simulink model "KINvasion"  (Simulink 7.5)
settings: Solver=ode4  SolverMode=SingleTasking  StartTime=0.0  StopTime=inf  FixedStep=0.0005  RelTol=1e-3
model workspace (MAT data in the model file):
  col_x = 1
  col_y = 2
  EnemyNumber = 1
  DifficultyNumber = 2
  BaseRegen = 1
  WindowMinX = 2
  WindowMaxX = 3
  WindowMinY = 4
  WindowMaxY = 5
  ForceSize = 6
  FireTorque = 7
  MoneyPerShip = 9
  StartingMoney = 10
  StompForce = 8
  BombSize = 11
  MoneyDrops = 4
  BossNumber = 3
  DemoMode : num (value not decoded)
StartFcn:
  |  warndlg('Dexterit-E models cannot run under simulation. Please compile your model and run it from within Dexterit-E.');set_param(gcs,'SimulationCommand','stop')
undefined symbols (not defined in the file or in its folder): Process_Video_CMD, Video
libraries: xpclib x5, General x3, KINARM_general x1, KINARM_EP_loads x1
(part 1 of 3)
CloseFcn:
  | rtwprivate ssgencode ModelCloseRequest b2lab2d
settings Model: Creator=Chris Grebeldinger  LastModifiedBy=BrainAdjust  ModifiedComment=chris -- Wed Feb 16 09:18:30 2005 -- Version 1.1384  ModifiedHistory=Feb 16/05 - Add error repeat, add offset ramp  ExtModeArmWhenConnect=off  ExtModeLogAll=off  BufferReuse=off
settings SolverCC: AutoInsertRateTranBlk=on
settings DataIOCC: LimitDataPoints=off  SaveOutput=off  SaveTime=off  SignalLoggingName=sigsOut
settings OptimizationCC: BlockReduction=off  BooleanDataType=off  OptimizeBlockIOStorage=off  BufferReuse=off  EnforceIntegerDowncast=off  ExpressionFolding=off  FoldNonRolledExpr=off  LocalBlockOutputs=off  InitFltsAndDblsToZero=on
settings DebuggingCC: SaveWithParameterizedLinksMsg=none  SignalResolutionControl=TryResolveAllWithWarning  SolverPrmCheckMsg=none  MultiTaskDSMMsg=warning  MultiTaskCondExecSysMsg=none  StrictBusMsg=Warning
settings HardwareCC: ProdIntDivRoundTo=Zero  ProdEndianess=LittleEndian  ProdHWDeviceType=Generic->32-bit x86 compatible  TargetHWDeviceType=32-bit Generic
settings RTWCC: SystemTargetFile=xpctarget.tlc  TemplateMakefile=xpc_default_tmf  Description=xPC Target  ProcessScript=xpctarget_make_rtw_hook  IncludeERTFirstTime=on  RTWCompilerOptimization=On
settings CodeAppCC: MaxIdLength=63
settings xpcTargetCC: TargetFcnLib=ansi_tfl_tmw.mat  TargetFunctionLibrary=ANSI_C  ERTCodeCoverageTool=None  ParMdlRefBuildCompliant=off  PortableWordSizes=off  xPCisDownloadable=off  xPCLoadParamSetFile=off

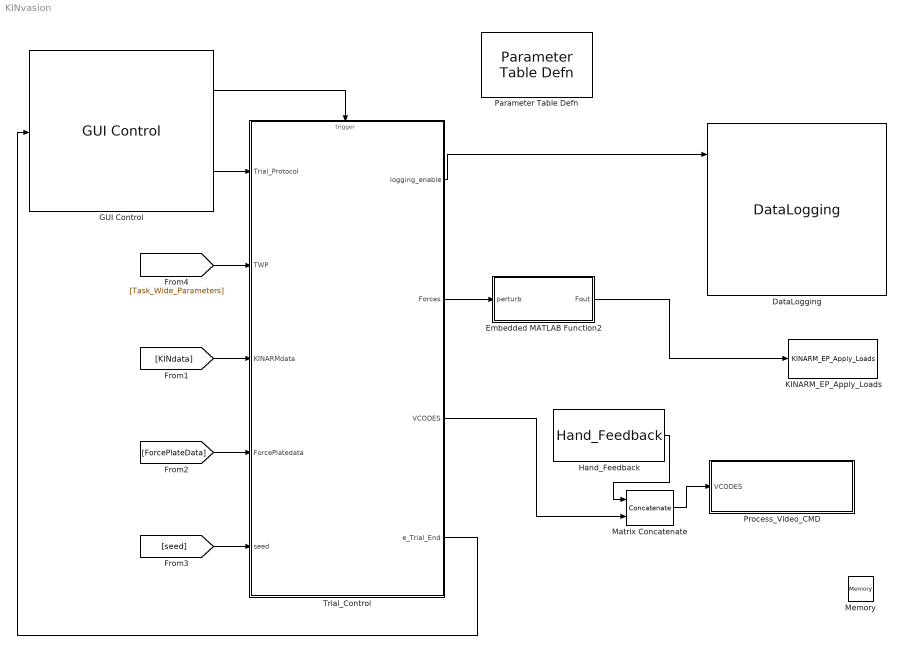
== system KINvasion ==
  DataLogging : General/DataLogging  SystemSampleTime=-1  log_event_codes=on  log_analog_inputs=on
      link override Poll KINARM/EPTorqueCMD: GotoTag=KINARMEPTorqueCMD
      link override Poll KINARM/TorqueCMD: GotoTag=KINARMTorqueCMD
  Embedded MATLAB Function2 : Stateflow chart  TreatAsAtomicUnit=on
  GUI Control : General/GUI Control  SystemSampleTime=-1  target_type_str=Circle  Target_Type=1  XYcols=[1 2]  Vcols=3  Lcols=4  indices_padding=[0 0 0 0;0 0 0 0]  task_version=1.0  show_repeat_trial_flag=off
  Hand_Feedback : KINARM_general/Hand_Feedback  SystemSampleTime=-1  feedback_cntl_src=none
  KINARM_EP_Apply_Loads : KINARM_EP_loads/KINARM_EP_Apply_Loads  SystemSampleTime=-1  up_duration=1500  down_duration=1500  max_force=30
  Matrix Concatenate : Concatenate  Mode=Multidimensional array
  Memory : Memory
  Parameter Table Defn : General/Parameter Table Defn  SystemSampleTime=-1  ShowInLibBrowser=0
  Process_Video_CMD : Subsystem  AncestorBlock=Video/Process_Video_CMD  LoadFcn=set_param(gcs, 'MaxIdLength', 63);  mask(Process_Video_CMD){}
      mask help:
      | <b>Do not rename this block, it must be called 'Process_Video_CMD'.</b>
      | <p>
      | This block takes a matrix of video commands (VCODES) as inputs (one VCODE per row) and processes them to display the appropriate video output.
      mask init:
      | block_path = gcb;  % store block path, as gcb may change with block operations
      | 
      | idxs = findstr(block_path, '/Process_Video_CMD');
      | [idxCount, n] = size(idxs);
      | [m, strlen] = size(block_path);
      | bColorSet = 0;
      | 
      | if idxCount == 0 || idxs(1) ~= strlen - 17
      |     fprintf('=========ERROR====================\n');
      |     fprintf('%s should be called Process_Video_CMD, attempting to rename.\n', block_path);
      |     try
      |         set_param(block_path, 'Name', 'Process_Video_CMD');
      |         block_path = gcb;  % store block path, as gcb may change with block operations
      |         fprintf('Rename successful\n');
      |     catch err
      |         fprintf('Rename failed. You may have 2 Process_Video_CMD blocks or another improperly named block.\n');
      |        	set_param(block_path, 'BackgroundColor', '[0.9, 0, 0]');
      |         bColorSet = 1;
      |     end
      |     fprintf('=============================\n');
      | end
      | 
      | 
      | % Handle background colours if link status changes.  If the link is resolved, 
      | % make the block back to the library colour.  If the link is not resolved, 
      | % change the colour to something other than the library block colour (but 
      | % only change it if it is the library colour, that way end-users can choose
      | % their own colour.
      | link_status = get_param(block_path, 'LinkStatus');
      | block_parent = get_param(block_path, 'Parent');
      | if bColorSet == 0 && (strcmp(link_status, 'resolved') || strcmp(block_parent, 'Video'))
      | 	set_param(block_path, 'BackgroundColor', '[0.85882, 0.69019, 0.3098]');
      | else
      |  	current_bgcolor = str2num( get_param(block_path, 'BackgroundColor') ) ;
      | 	%if the BackgroundColor is 'green', then after the str2num, current_bgcolor is empty
      | 	if ~isempty(current_bgcolor) 
      | 		if (round(current_bgcolor * 255) == [219 176 79])
      | 	 		set_param(block_path, 'BackgroundColor', 'green');
      | 		end
      | 	end
      | end
      mask Help:
      | Processes VCODES and sends a composite command over UDP to the GUI computer.
      | 
      | <H2>Library </H2>
      | Video
      | 
      | <H2>Description </H2>
      | <b>Do not rename this block, it must be called 'Process_Video_CMD'.</b>
      | <p>
      | The Process_Video_CMD block takes a matrix of video commands (VCODES) as inputs and processes them to display the appropriate video output.  The processed video command format is designed for use with GUI application.  There can be only one VCODE per row in the input.  To concatenate VCODEs properly prior to connecting a VCODE matrix to this block, the Matrix Concatenation block in the Simulink Math library should be used, with the concatenation method set to "Vertical".   For more information on the details of a VCODE, right click on the Show_Target block in the video library, click "Look Under Mask" and open the Embedded Matlab function.
      | <P>
      | The output command from this block is sent via UDP to an external computer for processing (note: this output is sent internally to the block - there is no output from the block that needs wiring to another block).
      | <P>
      | <B><I> There can be only one Process_Video_CMD block in a Task Program.</I></B>
      | 
      | <H2>Related Blocks </H2>
      | Show_Target<BR>
      | Show_Target_With_Label<BR>
      | Hand_Feedback<BR>
  Trial_Control : Stateflow chart  TreatAsAtomicUnit=on
  wires:
  GUI Control/2 -> Trial_Control/1(Trial_Protocol)
  GUI Control/1 -> Trial_Control/Trigger
  Trial_Control/1(logging_enable) -> DataLogging/1
  Trial_Control/4(e_Trial_End) -> GUI Control/1
  [Task_Wide_Parameters] -> Trial_Control/2(TWP)
  [KINdata] -> Trial_Control/3(KINARMdata)
  [seed] -> Trial_Control/5(seed)
  Trial_Control/3(VCODES) -> Matrix Concatenate/2
  Matrix Concatenate/1 -> Process_Video_CMD/1(VCODES)
  Hand_Feedback/1 -> Matrix Concatenate/1
  Embedded MATLAB Function2/1(Fout) -> KINARM_EP_Apply_Loads/1
  Trial_Control/2(Forces) -> Embedded MATLAB Function2/1(perturb)
  [ForcePlateData] -> Trial_Control/4(ForcePlatedata)

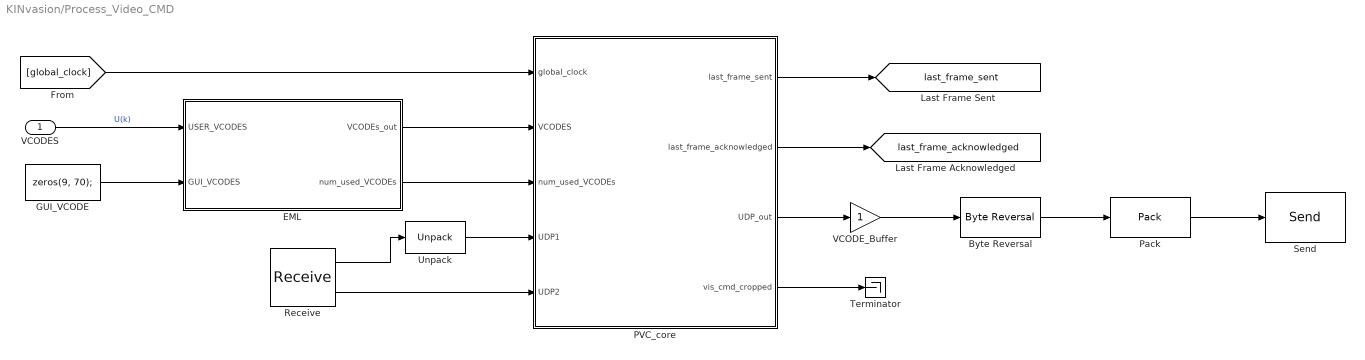
== system KINvasion/Process_Video_CMD ==
  VCODES : Inport  OutDataType=sfix(16)  OutScaling=2^0
  Byte Reversal : xpclib/UDP/Byte Reversal  numInp=1
  EML : Stateflow chart  TreatAsAtomicUnit=on
  GUI_VCODE : Constant  Value=zeros(9, 70);  VectorParams1D=off  OutDataTypeMode=double  OutDataType=sfix(16)  OutScaling=2^0  OutDataTypeStr=double
  PVC_core : Subsystem  TreatAsAtomicUnit=on
  Pack : xpclib/UDP/Pack  datatypes={'int32'}  byteAlign=1
  Receive : xpclib/UDP/Receive  ipAddress=192.168.0.1  ipPort=50002  width=4  vblLen=off  sampletime=0.001
  Send : xpclib/UDP/Send  ipAddress=192.168.0.1  ipPort=50002  localPort=50002  vblLen=off  sampletime=-1
  Terminator : Terminator
  Unpack : xpclib/UDP/Unpack  dimensions={[1]}  datatypes={'uint32'}  byteAlign=1
  VCODE_Buffer : Gain  ParameterDataType=sfix(16)  ParameterScaling=2^0  OutDataType=sfix(16)  OutScaling=2^0  SaturateOnIntegerOverflow=on  OutDataTypeStr=Inherit: Same as input  ParamDataTypeStr=Inherit: Same as input
  tag scope: last_frame_acknowledged=global, last_frame_sent=global
  wires:
  [global_clock] -> PVC_core/1(global_clock)
  PVC_core/2(last_frame_acknowledged) -> [last_frame_acknowledged]
  PVC_core/1(last_frame_sent) -> [last_frame_sent]
  VCODES/1 -> EML/1(USER_VCODES)  "U(k)"
  GUI_VCODE/1 -> EML/2(GUI_VCODES)
  EML/1(VCODEs_out) -> PVC_core/2(VCODES)
  EML/2(num_used_VCODEs) -> PVC_core/3(num_used_VCODEs)
  Receive/1 -> Unpack/1
  VCODE_Buffer/1 -> Byte Reversal/1
  Byte Reversal/1 -> Pack/1
  Pack/1 -> Send/1
  Unpack/1 -> PVC_core/4(UDP1)
  Receive/2 -> PVC_core/5(UDP2)
  PVC_core/3(UDP_out) -> VCODE_Buffer/1
  PVC_core/4(vis_cmd_cropped) -> Terminator/1

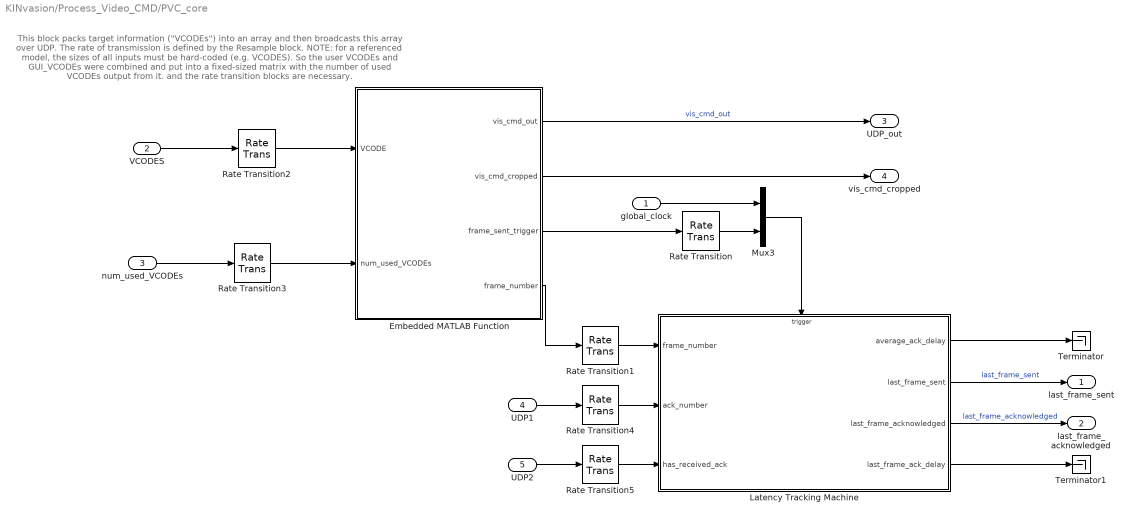
== system KINvasion/Process_Video_CMD/PVC_core ==
  note: This block packs target information ("VCODEs") into an array and then broadcasts this array over UDP. The rate of transmission is defined by the Resample block.
      |
      | NOTE: for a referenced model, the sizes of all inputs must be hard-coded (e.g. VCODES).  So the user VCODEs and GUI_VCODEs were combined and put into a fixed-sized
      | matrix with the number of used VCODEs output from it.    and the rate transition blocks are necessary.
  global_clock : Inport  PortDimensions=[1 1]  SampleTime=[0.00050000000000000001,0]  DataType=double  OutDataTypeStr=double
  VCODES : Inport  Port=2  PortDimensions=[89 70]  SampleTime=[0.00050000000000000001,0]  DataType=double  OutDataTypeStr=double
  num_used_VCODEs : Inport  Port=3  PortDimensions=1  SampleTime=[0.00050000000000000001,0]  DataType=double  OutDataTypeStr=double
  UDP1 : Inport  Port=4  PortDimensions=1  SampleTime=[0.001,0]  DataType=uint32  OutDataTypeStr=uint32
  UDP2 : Inport  Port=5  PortDimensions=1  SampleTime=[0.001,0]  DataType=double  OutDataTypeStr=double
  Embedded MATLAB Function : Stateflow chart  TreatAsAtomicUnit=on  SystemSampleTime=.002
  Latency Tracking Machine : Stateflow chart  TreatAsAtomicUnit=on
  Mux3 : Mux  Inputs=2
  Rate Transition{,1..5} (6 alike) : RateTransition
  Terminator : Terminator
  Terminator1 : Terminator
  last_frame_sent : Outport  PortDimensions=1  SampleTime=[0.00050000000000000001,0]  DataType=double  OutDataTypeStr=double
  last_frame_acknowledged : Outport  Port=2  PortDimensions=1  SampleTime=[0.00050000000000000001,0]  DataType=double  OutDataTypeStr=double
  UDP_out : Outport  Port=3  PortDimensions=725  SampleTime=[0.002,0]  DataType=int32  OutDataTypeStr=int32
  vis_cmd_cropped : Outport  Port=4  PortDimensions=1
  wires:
  Rate Transition5/1 -> Latency Tracking Machine/3(has_received_ack)
  Rate Transition4/1 -> Latency Tracking Machine/2(ack_number)
  UDP2/1 -> Rate Transition5/1
  UDP1/1 -> Rate Transition4/1
  Embedded MATLAB Function/1(vis_cmd_out) -> UDP_out/1  "vis_cmd_out"
  Rate Transition3/1 -> Embedded MATLAB Function/2(num_used_VCODEs)
  Rate Transition2/1 -> Embedded MATLAB Function/1(VCODE)
  num_used_VCODEs/1 -> Rate Transition3/1
  VCODES/1 -> Rate Transition2/1
  Rate Transition1/1 -> Latency Tracking Machine/1(frame_number)
  Rate Transition/1 -> Mux3/2
  Mux3/1 -> Latency Tracking Machine/Trigger
  Embedded MATLAB Function/4(frame_number) -> Rate Transition1/1
  Embedded MATLAB Function/3(frame_sent_trigger) -> Rate Transition/1
  Latency Tracking Machine/4(last_frame_ack_delay) -> Terminator1/1
  Latency Tracking Machine/1(average_ack_delay) -> Terminator/1
  global_clock/1 -> Mux3/1
  Latency Tracking Machine/2(last_frame_sent) -> last_frame_sent/1  "last_frame_sent"
  Latency Tracking Machine/3(last_frame_acknowledged) -> last_frame_acknowledged/1  "last_frame_acknowledged"
  Embedded MATLAB Function/2(vis_cmd_cropped) -> vis_cmd_cropped/1
